simulink model "VoltageDetection"  (R2024b)
settings: Solver=VariableStepAuto  StartTime=0.0  StopTime=2  RelTol=1e-3
undefined symbols (not defined in the file): HighVoltage, LowVoltage
settings Model: DataDictionary=VoltageDetection.sldd  Creator=User  LastModifiedBy=User

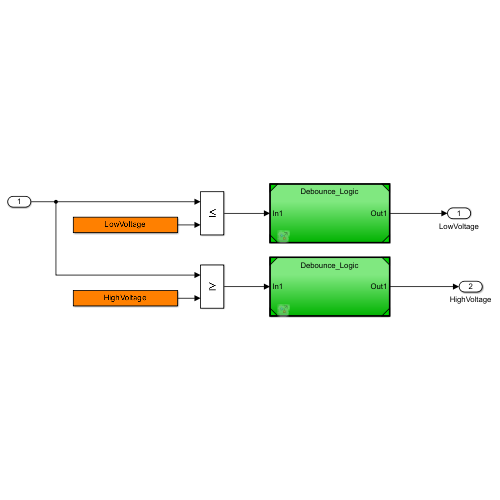
[thumbnail: Simulink's stored preview of the top-level diagram]
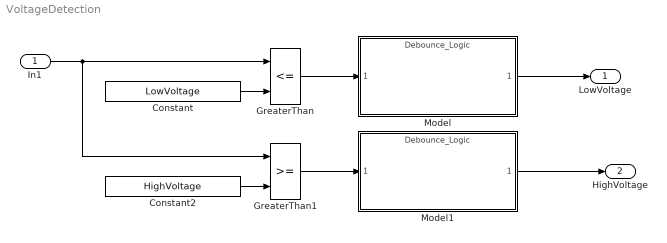
== system VoltageDetection ==
  In1 : Inport
  Constant : Constant  Value=LowVoltage
  Constant2 : Constant  Value=HighVoltage
  GreaterThan : RelationalOperator  Operator=<=  OutDataTypeStr=boolean  RndMeth=Simplest  InputSameDT=off
  GreaterThan1 : RelationalOperator  OutDataTypeStr=boolean  RndMeth=Simplest  InputSameDT=off
  Model : ModelReference  ModelNameDialog=Debounce_Logic.slx  SimulationMode=Normal  ModelReferenceVersion=1.11
  Model1 : ModelReference  ModelNameDialog=Debounce_Logic.slx  SimulationMode=Normal  ModelReferenceVersion=1.11
  LowVoltage : Outport
  HighVoltage : Outport  Port=2
  wires:
  Model/1 -> LowVoltage/1
  Model1/1 -> HighVoltage/1
  In1/1 -> GreaterThan/1, GreaterThan1/1
  GreaterThan/1 -> Model/1
  Constant/1 -> GreaterThan/2
  GreaterThan1/1 -> Model1/1
  Constant2/1 -> GreaterThan1/2
